simulink model "aero2_cascade_professor_format_report_experiment"  (R2024b)
settings: Solver=ode1  StartTime=0.0  StopTime=60  FixedStep=0.002  RelTol=1e-3
model workspace (MAT data in the model file):
  Kd = 3.88928113461
  Kff = 1
  Ki = 0
  Kp = 3.78162693601
  Ts = 0.002
  U_h = timeseries
  U_h.Name = 'unnamed'
  U_h.DataInfo = tsdata.datametadata
  U_h.DataInfo.Interpolation = tsdata.interpolation
  U_h.DataInfo.Interpolation.Fhandle : function handle (value not decoded)
  U_h.DataInfo.Interpolation.Name = 'linear'
  U_h.TimeInfo = tsdata.timemetadata
  U_h.TimeInfo.Length = 30001
  U_h.TimeInfo.DuplicateTimes = 0
  U_h.TimeInfo.Time_ = [0 0.002 0.004 0.006 0.008 0.01 0.012 0.014 0.016 0.018 0.02 0.022 ... (30001 elements, 30001x1)]
  U_h.TimeInfo.Initialized = 1
  U_h.QualityInfo = tsdata.qualmetadata
  U_h.Data_ = [0 0 0 0 0 0 0 0 0 0 0 0 ... (30001 elements, 30001x1)]
  U_v = timeseries
  U_v.Name = 'unnamed'
  U_v.DataInfo = tsdata.datametadata
  U_v.DataInfo.Interpolation = tsdata.interpolation
  U_v.DataInfo.Interpolation.Fhandle : function handle (value not decoded)
  U_v.DataInfo.Interpolation.Name = 'linear'
  U_v.TimeInfo = tsdata.timemetadata
  U_v.TimeInfo.Length = 30001
  U_v.TimeInfo.DuplicateTimes = 0
  U_v.TimeInfo.Time_ = [0 0.002 0.004 0.006 0.008 0.01 0.012 0.014 0.016 0.018 0.02 0.022 ... (30001 elements, 30001x1)]
  U_v.TimeInfo.Initialized = 1
  U_v.QualityInfo = tsdata.qualmetadata
  U_v.Data_ = [0 0 0 0 0 0 0 0 0 0 0 0 ... (30001 elements, 30001x1)]
  ki_PI_motor = 1.84164606325
  kp_PI_motor = 0.216370391856
  kw_PI_motor = 10.85985
  meas_on = 1
  tmax = 60
Description:
  | Lab 2 nominal PD + exact inverse + IP cascade in the professor layout.
  | Visible +/-24 V limits feed both the plant and IP anti-windup ports.
  | Kp=3.7816, Kd=3.8893, Ki=0; motor Kp=0.2164, Ki=1.8416, Kaw=20.0000.
  | Original smooth course references; sensor effects on; tachometer LPFs 180 rad/s.
settings Model: ExtModeTrigDuration=20000  Creator=MLevis  LastModifiedBy=matiasgarcia
settings DebuggingCC: UnderspecifiedInitializationDetection=Classic  MergeDetectMultiDrivingBlocksExec=none
settings ModelReferenceCC: PropagateSignalLabelsOutOfModel=off

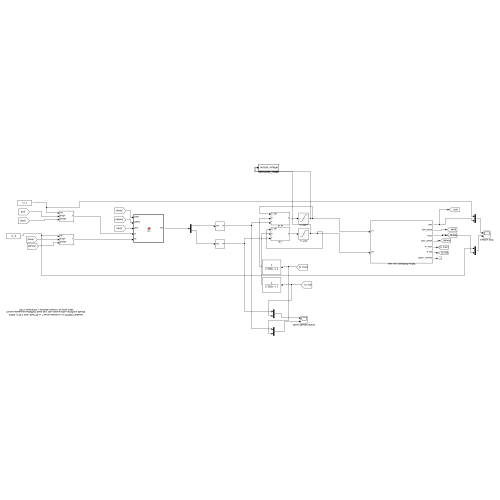
[thumbnail: Simulink's stored preview of the top-level diagram]
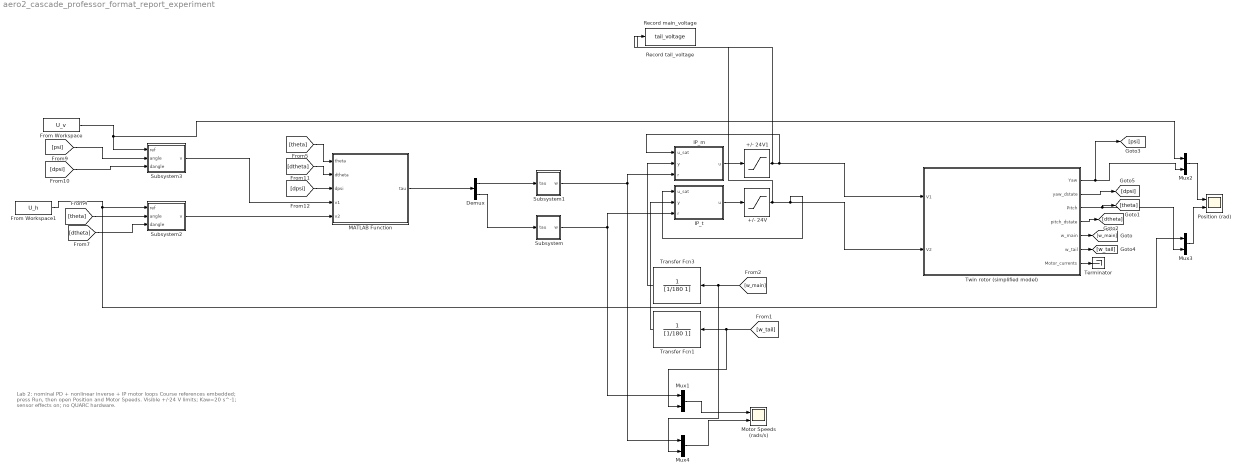
== system aero2_cascade_professor_format_report_experiment ==
  note: Lab 2: nominal PD + nonlinear inverse + IP motor loops
      | Course references embedded; press Run, then open Position and Motor Speeds.
      | Visible +/-24 V limits; Kaw=20 s^-1; sensor effects on; no QUARC hardware.
  +/- 24V : Saturate  UpperLimit=24  LowerLimit=-24
  +/- 24V1 : Saturate  UpperLimit=24  LowerLimit=-24
  Demux : Demux  Outputs=2
  From Workspace : FromWorkspace  VariableName=U_v  OutputAfterFinalValue=Setting to zero
  From Workspace1 : FromWorkspace  VariableName=U_h  OutputAfterFinalValue=Setting to zero
  IP_m : Subsystem
  IP_t : Subsystem
  MATLAB Function : MATLAB Function  TreatAsAtomicUnit=on
  Motor Speeds (rads/s) : Scope  NumInputPorts=2
  Mux{1..4} (4 alike) : Mux  Inputs=2
  Position (rad) : Scope  NumInputPorts=2
  Record main_voltage : ToWorkspace  VariableName=main_voltage  SaveFormat=Timeseries  SampleTime=-1
  Record tail_voltage : ToWorkspace  VariableName=tail_voltage  SaveFormat=Timeseries  SampleTime=-1
  Subsystem : Subsystem
  Subsystem1 : Subsystem
  Subsystem2 : Subsystem
  Subsystem3 : Subsystem
  Terminator : Terminator
  Transfer Fcn1 : TransferFcn  Denominator=[1/180 1]
  Transfer Fcn3 : TransferFcn  Denominator=[1/180 1]
  Twin rotor (simplified model) : Subsystem  mask{meas=meas_on}
      mask prompts: meas "Measurement effects (1 = encoder quantization + sensor noise, 0 = ideal)"
      mask help: Simplified twin-rotor model (eq. (simp) of twin_rotor_FL_merged.tex) with DC-motor rotor dynamics. Inputs: V1 main-rotor voltage, V2 tail-rotor voltage [V]. Outputs: same signals as the QUARC interface of lin_feedback_v1.slx, continuous (no zero-order holds; sensor noise generated at Ts).
  wires:
  +/- 24V/1 -> IP_t/1(u_sat), Twin rotor (simplified model)/2(V2), Record tail_voltage/1
  +/- 24V1/1 -> IP_m/1(u_sat), Twin rotor (simplified model)/1(V1), Record main_voltage/1
  IP_m/1(u) -> +/- 24V1/1
  IP_t/1(u) -> +/- 24V/1
  Mux1/1 -> Motor Speeds (rads/s)/1
  Mux4/1 -> Motor Speeds (rads/s)/2
  [w_main] -> Mux4/2, Transfer Fcn3/1
  [w_tail] -> Mux1/2, Transfer Fcn1/1
  Subsystem1/1(w) -> IP_m/3(r), Mux4/1
  Transfer Fcn3/1 -> IP_m/2(y)
  Subsystem/1(w) -> IP_t/3(r), Mux1/1
  Transfer Fcn1/1 -> IP_t/2(y)
  [theta] -> Subsystem2/2(angle)
  [dtheta] -> Subsystem2/3(dangle)
  [psi] -> Subsystem3/2(angle)
  [dpsi] -> Subsystem3/3(dangle)
  Subsystem3/1(v) -> MATLAB Function/4(v1)
  Subsystem2/1(v) -> MATLAB Function/5(v2)
  From Workspace1/1 -> Subsystem2/1(ref), Mux3/1
  From Workspace/1 -> Subsystem3/1(ref), Mux2/1
  Mux2/1 -> Position (rad)/1
  Mux3/1 -> Position (rad)/2
  [theta] -> MATLAB Function/1(theta)
  [dtheta] -> MATLAB Function/2(dtheta)
  [dpsi] -> MATLAB Function/3(dpsi)
  Demux/1 -> Subsystem1/1(tau)
  Demux/2 -> Subsystem/1(tau)
  MATLAB Function/1(tau) -> Demux/1
  Twin rotor (simplified model)/7(Motor_currents) -> Terminator/1
  Twin rotor (simplified model)/3(Pitch) -> [theta], Mux3/2
  Twin rotor (simplified model)/1(Yaw) -> [psi], Mux2/2
  Twin rotor (simplified model)/4(pitch_dstate) -> [dtheta]
  Twin rotor (simplified model)/5(w_main) -> [w_main]
  Twin rotor (simplified model)/6(w_tail) -> [w_tail]
  Twin rotor (simplified model)/2(yaw_dstate) -> [dpsi]

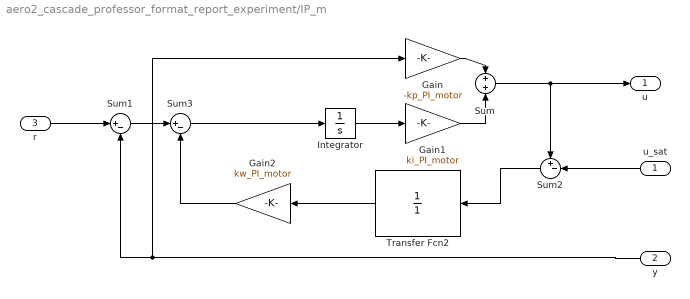
== system aero2_cascade_professor_format_report_experiment/IP_m ==
  u_sat : Inport
  y : Inport  Port=2
  r : Inport  Port=3
  Gain : Gain  Gain=-kp_PI_motor
  Gain1 : Gain  Gain=ki_PI_motor
  Gain2 : Gain  Gain=kw_PI_motor
  Integrator : Integrator
  Sum : Sum  Inputs=+|+
  Sum1 : Sum  Inputs=|+-
  Sum2 : Sum  Inputs=+-|
  Sum3 : Sum  Inputs=|+-
  Transfer Fcn2 : TransferFcn  Numerator=1  Denominator=1
  u : Outport
  wires:
  Integrator/1 -> Gain1/1
  Gain/1 -> Sum/1
  Sum/1 -> u/1, Sum2/1
  y/1 -> Gain/1, Sum1/2
  Sum2/1 -> Transfer Fcn2/1
  Gain1/1 -> Sum/2
  Sum1/1 -> Sum3/1
  Transfer Fcn2/1 -> Gain2/1
  Gain2/1 -> Sum3/2
  Sum3/1 -> Integrator/1
  r/1 -> Sum1/1
  u_sat/1 -> Sum2/2

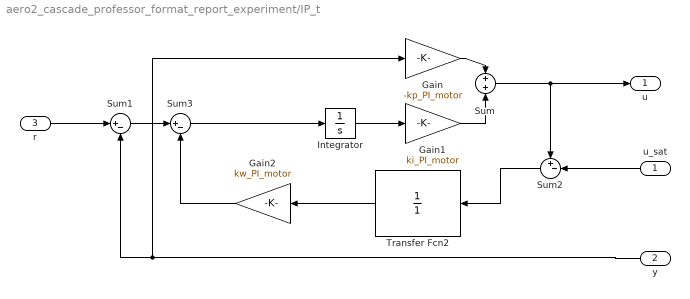
== system aero2_cascade_professor_format_report_experiment/IP_t ==
  u_sat : Inport
  y : Inport  Port=2
  r : Inport  Port=3
  Gain : Gain  Gain=-kp_PI_motor
  Gain1 : Gain  Gain=ki_PI_motor
  Gain2 : Gain  Gain=kw_PI_motor
  Integrator : Integrator
  Sum : Sum  Inputs=+|+
  Sum1 : Sum  Inputs=|+-
  Sum2 : Sum  Inputs=+-|
  Sum3 : Sum  Inputs=|+-
  Transfer Fcn2 : TransferFcn  Numerator=1  Denominator=1
  u : Outport
  wires:
  Integrator/1 -> Gain1/1
  Gain/1 -> Sum/1
  Sum/1 -> u/1, Sum2/1
  y/1 -> Gain/1, Sum1/2
  Sum2/1 -> Transfer Fcn2/1
  Gain1/1 -> Sum/2
  Sum1/1 -> Sum3/1
  Transfer Fcn2/1 -> Gain2/1
  Gain2/1 -> Sum3/2
  Sum3/1 -> Integrator/1
  r/1 -> Sum1/1
  u_sat/1 -> Sum2/2

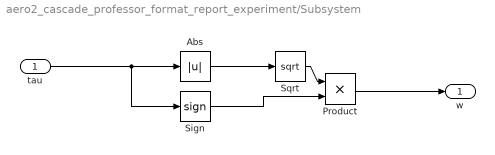
== system aero2_cascade_professor_format_report_experiment/Subsystem ==
  tau : Inport
  Abs : Abs  SaturateOnIntegerOverflow=off
  Product : Product
  Sign : Signum
  Sqrt : Sqrt
  w : Outport
  wires:
  tau/1 -> Sign/1, Abs/1
  Product/1 -> w/1
  Abs/1 -> Sqrt/1
  Sqrt/1 -> Product/1
  Sign/1 -> Product/2

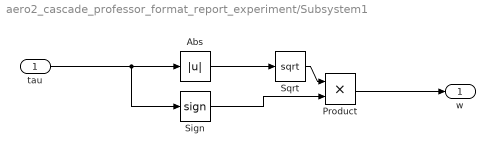
== system aero2_cascade_professor_format_report_experiment/Subsystem1 ==
  tau : Inport
  Abs : Abs  SaturateOnIntegerOverflow=off
  Product : Product
  Sign : Signum
  Sqrt : Sqrt
  w : Outport
  wires:
  tau/1 -> Sign/1, Abs/1
  Product/1 -> w/1
  Abs/1 -> Sqrt/1
  Sqrt/1 -> Product/1
  Sign/1 -> Product/2

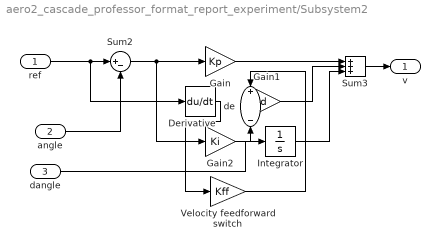
== system aero2_cascade_professor_format_report_experiment/Subsystem2 ==
  ref : Inport
  angle : Inport  Port=2
  dangle : Inport  Port=3
  Derivative : Derivative
  Gain : Gain  Gain=Kp
  Gain1 : Gain  Gain=Kd
  Gain2 : Gain  Gain=Ki
  Integrator : Integrator
  Sum2 : Sum  Inputs=|+-
  Sum3 : Sum  Inputs=+++
  Velocity feedforward switch : Gain  Gain=Kff
  de : Sum  Description=Kd term: d(ref)/dt - measured rate (no derivative of the quantized error)  Inputs=+-
  v : Outport
  wires:
  Sum2/1 -> Gain/1, Gain2/1
  Gain/1 -> Sum3/1
  ref/1 -> Sum2/1, Derivative/1
  Gain1/1 -> Sum3/2
  angle/1 -> Sum2/2
  Sum3/1 -> v/1
  Gain2/1 -> Integrator/1
  Integrator/1 -> Sum3/3
  Derivative/1 -> Velocity feedforward switch/1
  dangle/1 -> de/2
  de/1 -> Gain1/1
  Velocity feedforward switch/1 -> de/1

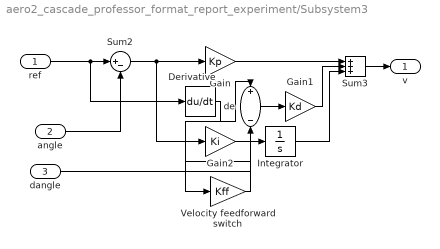
== system aero2_cascade_professor_format_report_experiment/Subsystem3 ==
  ref : Inport
  angle : Inport  Port=2
  dangle : Inport  Port=3
  Derivative : Derivative
  Gain : Gain  Gain=Kp
  Gain1 : Gain  Gain=Kd
  Gain2 : Gain  Gain=Ki
  Integrator : Integrator
  Sum2 : Sum  Inputs=|+-
  Sum3 : Sum  Inputs=+++
  Velocity feedforward switch : Gain  Gain=Kff
  de : Sum  Description=Kd term: d(ref)/dt - measured rate (no derivative of the quantized error)  Inputs=+-
  v : Outport
  wires:
  Sum2/1 -> Gain/1, Gain2/1
  Gain/1 -> Sum3/1
  ref/1 -> Sum2/1, Derivative/1
  Gain1/1 -> Sum3/2
  angle/1 -> Sum2/2
  Sum3/1 -> v/1
  Gain2/1 -> Integrator/1
  Integrator/1 -> Sum3/3
  Derivative/1 -> Velocity feedforward switch/1
  dangle/1 -> de/2
  de/1 -> Gain1/1
  Velocity feedforward switch/1 -> de/1

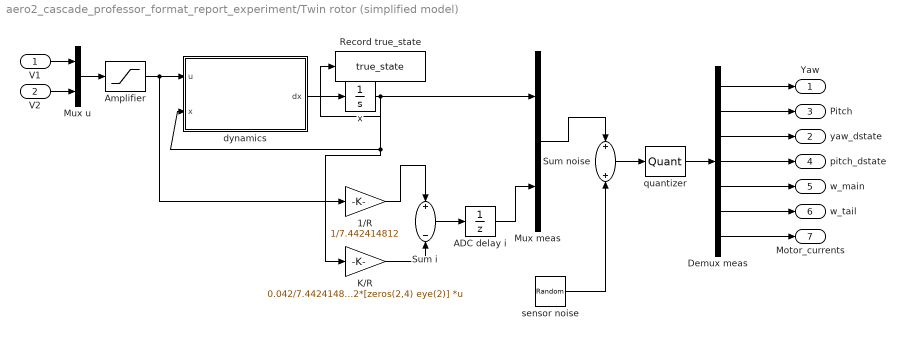
== system aero2_cascade_professor_format_report_experiment/Twin rotor (simplified model) ==
  V1 : Inport
  V2 : Inport  Port=2
  1/R : Gain  Gain=1/7.442414812
  ADC delay i : UnitDelay  InitialCondition=[0;0]  SampleTime=0.002  HasFrameUpgradeWarning=on
  Amplifier : Saturate  UpperLimit=24  LowerLimit=-24
  Demux meas : Demux  Outputs=[1 1 1 1 1 1 2]
  K/R : Gain  Gain=0.042/7.442414812*[zeros(2,4) eye(2)]  Multiplication=Matrix(K*u)
  Mux meas : Mux  Inputs=[6 2]
  Mux u : Mux  Inputs=2
  Record true_state : ToWorkspace  VariableName=true_state  SaveFormat=Timeseries  SampleTime=-1
  Sum i : Sum  Inputs=+-
  Sum noise : Sum
  dynamics : MATLAB Function  TreatAsAtomicUnit=on
  quantizer : Quantizer  QuantizationInterval=max((meas)*[0.0015339807878856412;0.0030679615757712823;0.001;0.001;0.050000000000000003;0.050000000000000003;0.001;0.001], 1e-12)
  sensor noise : RandomNumber  Mean=zeros(8,1)  Variance=((meas)*[0.0005;0.0005;0.005;0.005;0.3;0.3;0.01;0.01]).^2  Seed=[61027;18839;4421;30893;23341;7781;51117;9013]  SampleTime=0.002
  x : Integrator  InitialCondition=zeros(6,1)
  Yaw : Outport
  yaw_dstate : Outport  Port=2
  Pitch : Outport  Port=3
  pitch_dstate : Outport  Port=4
  w_main : Outport  Port=5
  w_tail : Outport  Port=6
  Motor_currents : Outport  Port=7
  wires:
  V1/1 -> Mux u/1
  V2/1 -> Mux u/2
  Mux u/1 -> Amplifier/1
  Amplifier/1 -> dynamics/1(u), 1/R/1
  dynamics/1(dx) -> x/1
  x/1 -> Mux meas/1, dynamics/2(x), K/R/1, Record true_state/1
  1/R/1 -> Sum i/1
  K/R/1 -> Sum i/2
  Sum i/1 -> ADC delay i/1
  ADC delay i/1 -> Mux meas/2
  Mux meas/1 -> Sum noise/1
  sensor noise/1 -> Sum noise/2
  Sum noise/1 -> quantizer/1
  quantizer/1 -> Demux meas/1
  Demux meas/1 -> Yaw/1
  Demux meas/3 -> yaw_dstate/1
  Demux meas/2 -> Pitch/1
  Demux meas/4 -> pitch_dstate/1
  Demux meas/5 -> w_main/1
  Demux meas/6 -> w_tail/1
  Demux meas/7 -> Motor_currents/1

== matlab function aero2_cascade_professor_format_report_experiment/Twin rotor (simplified model)/dynamics ==
  data: u input; dx output; x input
function dx = fcn(u, x)
%% Simplified twin-rotor model of aero2_model.pdf (2-DOF body + first-order motors)
p = struct('Jph', 0.64070000000000005, ...
    'jph', 0.01, ...
    'Jth', 0.71640000000000004, ...
    'G', 0.025399999999999999, ...
    'kT', 4.2486999999999997e-06, ...
    'kF', 2.5525999999999999e-05, ...
    'L', 0.16700000000000001, ...
    'Cor', 0.63070000000000004, ...
    'Dph', 0, ...
    'Dth', 0, ...
    'aw', 5.7800000000000002, ...
    'bw', 96.531999999999996);
dx = tr_simp_dyn(x, u, p);
end

function dx = tr_simp_dyn(x, u, p)
%TR_SIMP_DYN  Simplified twin-rotor model with voltage inputs (aero2_model.pdf).
%   Body: reduced 2-DOF model, eq. (simp) of twin_rotor_FL_merged.tex
%     Mq(th) [ddpsi; ddth] + cq + Bq dq + gq = Gamma(th) [wm|wm|; wt|wt|]
%   with cq = [-Cor sin(2th) dth dpsi; 1/2 Cor sin(2th) dpsi^2]
%   (no gyroscopic coupling, no motor reaction channel, s_m=+1, s_t=-1).
%   Rotors: first-order motor model of the hand-out
%     dw = -aw w + bw v
%   State x = [psi, theta, dpsi, dtheta, wm, wt], input u = [Um, Ut].
%   p: Jph jph Jth Dph Dth Cor L G kF kT aw bw (psim of tr_instructor_params).
%   Codegen-compatible (used inside the Simulink MATLAB Function plant block).

    th = x(2);  dps = x(3);  dth = x(4);
    c = cos(th);  s = sin(th);
    tau = [x(5)*abs(x(5)); x(6)*abs(x(6))];

    Ms  = [p.Jph*c^2 + p.jph*s^2, 0; 0, p.Jth];
    Cs  = [-p.Cor*sin(2*th)*dth*dps; 0.5*p.Cor*sin(2*th)*dps^2];
    Ds  = [p.Dph*dps; p.Dth*dth];
    Gs  = [0; p.G*s];
    Gam = [c 0; 0 1]*[-p.kT, p.L*p.kF; p.L*p.kF, p.kT];
    ddq = Ms\(Gam*tau - Cs - Ds - Gs);

    dw  = -p.aw*x(5:6) + p.bw*u(:);
    dx  = [x(3:4); ddq; dw];
end

== matlab function aero2_cascade_professor_format_report_experiment/MATLAB Function ==
  data: theta input; tau output; dtheta input; dpsi input; v1 input; v2 input
function tau = fcn(theta,dtheta,dpsi,v1,v2)

Jph = 0.6407;
jph = 0.01;
Jth = 0.7164;
Dph = 0;          % B_q = 0 (aero2_model.pdf)
Dth = 0;
Cor = Jph - jph;

L = 0.167;
G = 0.0254;
kF=2.5526e-5;
kT=4.2487e-6;

M=[Jph*cos(theta)^2+jph*sin(theta)^2,0;
    0, Jth    ];
C=[-Cor*sin(2*theta)*dtheta*dpsi;
    (1/2)*Cor*sin(2*theta)*dpsi^2
  %  (1/2)*Cor*(2*theta)*dpsi^2
    ];

D=[Dph*dpsi;Dth*dtheta];

Grav=[0;
    G*sin(theta)];
Gamma=[cos(theta),0;0,1]*[-kT,L*kF;L*kF,kT];

den=L*L*kF*kF+kT*kT;
Gamma_inv=(1/den)*[-kT,L*kF;L*kF,kT]*[1/cos(theta),0;0,1];

v=[v1(1,1);v2(1,1)];

%tau=inv(Gamma)*(M*v+C+Grav);
tau=Gamma_inv*(M*v+C+D+Grav);
